simulink model "can2_mcu_power_pack"  (R2026b)
settings: Solver=VariableStepAuto
undefined symbols (not defined in the file or in its folder): P
libraries: simulink x1, svdutilitieslib x1
settings Model: Creator=aomar  LastModifiedBy=aomar

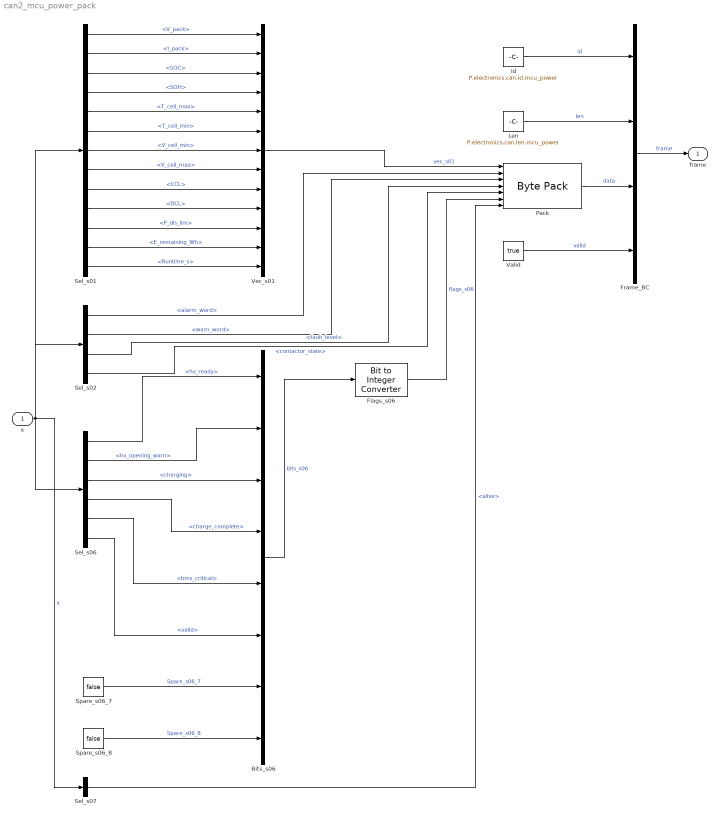
== system can2_mcu_power_pack ==
  x : Inport  OutDataTypeStr=Bus: Bus_BmsStatus
  Bits_s06 : Concatenate  NumInputs=8
  Flags_s06 : simulink/Logic and Bit Operations/Bit to Integer Converter  nbits=8  bitOrder=LSB first  signedOutputValues=Unsigned  outDtype=uint8  outDtypeSigned=Inherit via internal rule
      settings: LibrarySourceBlock=|
      | commutil2/Bit to Integer
      | Converter
  Frame_BC : BusCreator  Inputs=4  OutDataTypeStr=Bus: Bus_CanFrame64  NonVirtualBus=on
      settings: InheritFromInputs=off
  Id : Constant  Value=P.electronics.can.id.mcu_power  OutDataTypeStr=uint32  SampleTime=-1
  Len : Constant  Value=P.electronics.can.len.mcu_power  OutDataTypeStr=uint8  SampleTime=-1
  Pack : svdutilitieslib/Byte Pack  maskPackedDataType=uint8  datatypes={'single','uint32','uint32','uint8','uint8','uint8','uint8'}  byteAlign=1  blockPlatform=arduinoert
      settings: LibrarySourceBlock=mcblib/Signal Management/Byte Pack
  Sel_s01 : BusSelector  OutputSignals=V_pack,I_pack,SOC,SOH,T_cell_max,T_cell_min,V_cell_min,V_cell_max,CCL,DCL,P_dis_lim,E_remaining_Wh,Runtime_s
  Sel_s02 : BusSelector  OutputSignals=alarm_word,warn_word,fault_level,contactor_state
  Sel_s06 : BusSelector  OutputSignals=hv_ready,hv_opening_warn,charging,charge_complete,bms_critical,valid
  Sel_s07 : BusSelector  OutputSignals=alive
  Spare_s06_7 : Constant  Value=false  OutDataTypeStr=boolean  SampleTime=-1
  Spare_s06_8 : Constant  Value=false  OutDataTypeStr=boolean  SampleTime=-1
  Valid : Constant  Value=true  OutDataTypeStr=boolean  SampleTime=-1
  Vec_s01 : Concatenate  NumInputs=13
  frame : Outport  OutDataTypeStr=Bus: Bus_CanFrame64
  wires:
  x/1 -> Sel_s07/1, Sel_s01/1, Sel_s02/1, Sel_s06/1  "x"
  Sel_s01/1 -> Vec_s01/1  "<V_pack>"
  Sel_s01/2 -> Vec_s01/2  "<I_pack>"
  Sel_s01/3 -> Vec_s01/3  "<SOC>"
  Sel_s01/4 -> Vec_s01/4  "<SOH>"
  Sel_s01/5 -> Vec_s01/5  "<T_cell_max>"
  Sel_s01/6 -> Vec_s01/6  "<T_cell_min>"
  Sel_s01/7 -> Vec_s01/7  "<V_cell_min>"
  Sel_s01/8 -> Vec_s01/8  "<V_cell_max>"
  Sel_s01/9 -> Vec_s01/9  "<CCL>"
  Sel_s01/10 -> Vec_s01/10  "<DCL>"
  Sel_s01/11 -> Vec_s01/11  "<P_dis_lim>"
  Sel_s01/12 -> Vec_s01/12  "<E_remaining_Wh>"
  Sel_s01/13 -> Vec_s01/13  "<Runtime_s>"
  Sel_s02/1 -> Pack/2  "<alarm_word>"
  Sel_s02/2 -> Pack/3  "<warn_word>"
  Sel_s02/3 -> Pack/4  "<fault_level>"
  Sel_s02/4 -> Pack/5  "<contactor_state>"
  Sel_s06/1 -> Bits_s06/1  "<hv_ready>"
  Sel_s06/2 -> Bits_s06/2  "<hv_opening_warn>"
  Sel_s06/3 -> Bits_s06/3  "<charging>"
  Sel_s06/4 -> Bits_s06/4  "<charge_complete>"
  Sel_s06/5 -> Bits_s06/5  "<bms_critical>"
  Sel_s06/6 -> Bits_s06/6  "<valid>"
  Sel_s07/1 -> Pack/7  "<alive>"
  Spare_s06_7/1 -> Bits_s06/7  "Spare_s06_7"
  Spare_s06_8/1 -> Bits_s06/8  "Spare_s06_8"
  Vec_s01/1 -> Pack/1  "vec_s01"
  Bits_s06/1 -> Flags_s06/1  "bits_s06"
  Flags_s06/1 -> Pack/6  "flags_s06"
  Id/1 -> Frame_BC/1  "id"
  Len/1 -> Frame_BC/2  "len"
  Valid/1 -> Frame_BC/4  "valid"
  Pack/1 -> Frame_BC/3  "data"
  Frame_BC/1 -> frame/1  "frame"
